simulink model "AFS_FinTabSim"  (R2026a)
settings: Solver=ode45  StopTime=P.sim.tStop  MaxStep=P.sim.maxStep  RelTol=1e-5
PostLoadFcn:
  | addpath(fileparts(get_param('AFS_FinTabSim','FileName')));
  | if ~evalin('base','exist(''P'',''var'')'), assignin('base','P',afs_params()); end
InitFcn:
  | if ~exist('P','var'), P = afs_params(); end
values from neighbouring files (symbols this model uses):
  P = afs_params()    [build_AFS_FinTabSim.m]    (also in run_AFS_FinTabSim.m)
libraries: simulink x4
settings Model: Creator=lando  LastModifiedBy=lando

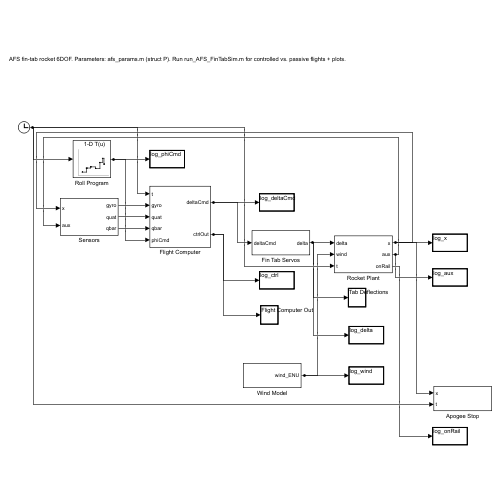
[thumbnail: Simulink's stored preview of the top-level diagram]
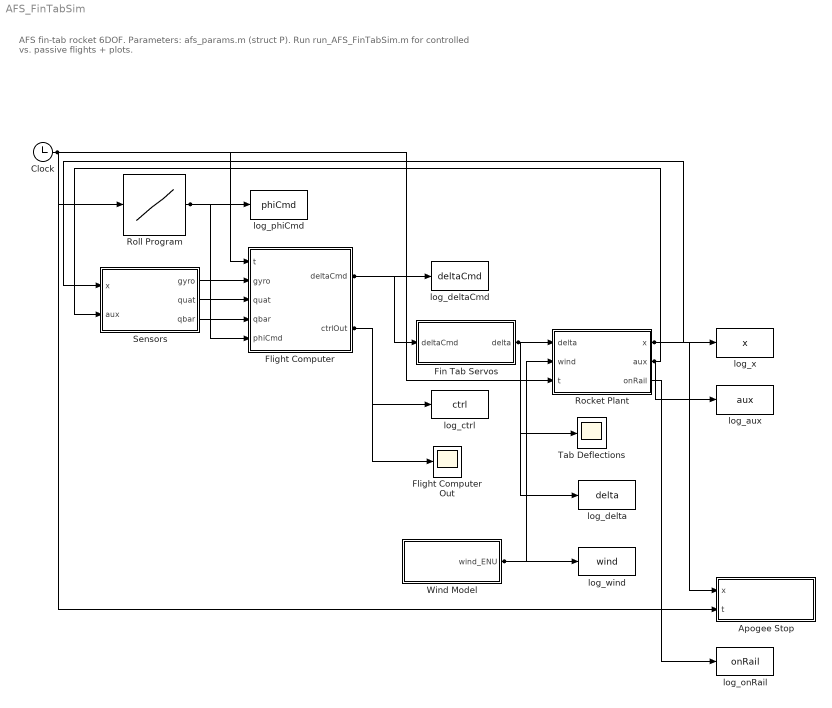
== system AFS_FinTabSim ==
  note: AFS fin-tab rocket 6DOF. Parameters: afs_params.m (struct P). Run run_AFS_FinTabSim.m for controlled vs. passive flights + plots.
  Apogee Stop : Subsystem
  Clock : Clock
  Fin Tab Servos : Subsystem
  Flight Computer : Subsystem
  Flight Computer Out : Scope
  Rocket Plant : Subsystem
  Roll Program : Lookup_n-D  NumberOfTableDimensions=1  BreakpointsForDimension1=P.ctrl.rollProg.t  Table=P.ctrl.rollProg.phi  InterpMethod=Flat  ExtrapMethod=Clip  InternalRulePriority=Speed  RndMeth=Simplest
  Sensors : Subsystem
  Tab Deflections : Scope
  Wind Model : Subsystem
  log_aux : ToWorkspace  VariableName=aux  SaveFormat=Timeseries  SampleTime=-1
  log_ctrl : ToWorkspace  VariableName=ctrl  SaveFormat=Timeseries  SampleTime=-1
  log_delta : ToWorkspace  VariableName=delta  SaveFormat=Timeseries  SampleTime=-1
  log_deltaCmd : ToWorkspace  VariableName=deltaCmd  SaveFormat=Timeseries  SampleTime=-1
  log_onRail : ToWorkspace  VariableName=onRail  SaveFormat=Timeseries  SampleTime=-1
  log_phiCmd : ToWorkspace  VariableName=phiCmd  SaveFormat=Timeseries  SampleTime=-1
  log_wind : ToWorkspace  VariableName=wind  SaveFormat=Timeseries  SampleTime=-1
  log_x : ToWorkspace  VariableName=x  SaveFormat=Timeseries  SampleTime=-1
  wires:
  Clock/1 -> Rocket Plant/3(t), Flight Computer/1(t), Apogee Stop/2(t), Roll Program/1
  Rocket Plant/3(onRail) -> log_onRail/1
  Roll Program/1 -> Flight Computer/5(phiCmd), log_phiCmd/1
  Sensors/3(qbar) -> Flight Computer/4(qbar)
  Sensors/2(quat) -> Flight Computer/3(quat)
  Sensors/1(gyro) -> Flight Computer/2(gyro)
  Flight Computer/2(ctrlOut) -> log_ctrl/1, Flight Computer Out/1
  Flight Computer/1(deltaCmd) -> Fin Tab Servos/1(deltaCmd), log_deltaCmd/1
  Fin Tab Servos/1(delta) -> Rocket Plant/1(delta), log_delta/1, Tab Deflections/1
  Wind Model/1(wind_ENU) -> Rocket Plant/2(wind), log_wind/1
  Rocket Plant/1(x) -> Apogee Stop/1(x), Sensors/1(x), log_x/1
  Rocket Plant/2(aux) -> Sensors/2(aux), log_aux/1

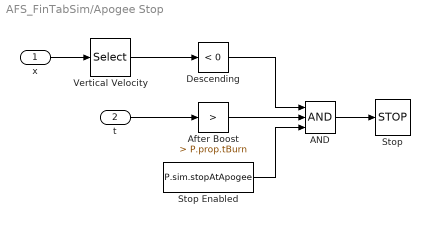
== system AFS_FinTabSim/Apogee Stop ==
  x : Inport
  t : Inport  Port=2
  AND : Logic  Inputs=3  AllPortsSameDT=off  OutDataTypeStr=boolean
  After Boost : simulink/Logic and Bit Operations/Compare To Constant  relop=>  const=P.prop.tBurn  OutDataTypeStr=boolean
  Descending : simulink/Logic and Bit Operations/Compare To Constant  relop=<  const=0  OutDataTypeStr=boolean
  Stop : Stop
  Stop Enabled : Constant  Value=P.sim.stopAtApogee  OutDataTypeStr=boolean
  Vertical Velocity : Selector  InputPortWidth=13  IndexOptions=Index vector (dialog)  Indices=6  OutputSizes=1
  wires:
  t/1 -> After Boost/1
  Vertical Velocity/1 -> Descending/1
  x/1 -> Vertical Velocity/1
  After Boost/1 -> AND/2
  Descending/1 -> AND/1
  AND/1 -> Stop/1
  Stop Enabled/1 -> AND/3

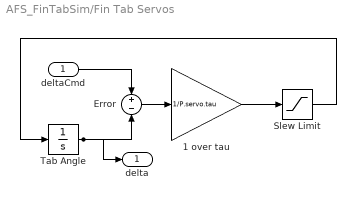
== system AFS_FinTabSim/Fin Tab Servos ==
  deltaCmd : Inport
  1 over tau : Gain  Gain=1/P.servo.tau
  Error : Sum  Inputs=+-
  Slew Limit : Saturate  UpperLimit=P.servo.rateMax  LowerLimit=-P.servo.rateMax
  Tab Angle : Integrator  InitialCondition=zeros(P.geo.nFins,1)  LimitOutput=on  UpperSaturationLimit=P.servo.defMax  LowerSaturationLimit=-P.servo.defMax
  delta : Outport
  wires:
  deltaCmd/1 -> Error/1
  Slew Limit/1 -> Tab Angle/1
  1 over tau/1 -> Slew Limit/1
  Tab Angle/1 -> Error/2, delta/1
  Error/1 -> 1 over tau/1

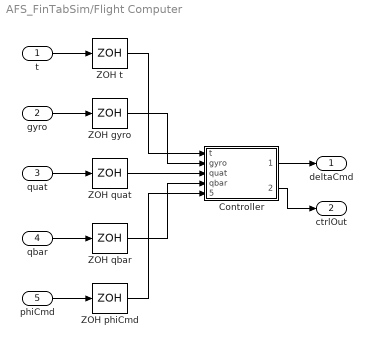
== system AFS_FinTabSim/Flight Computer ==
  t : Inport
  gyro : Inport  Port=2
  quat : Inport  Port=3
  qbar : Inport  Port=4
  phiCmd : Inport  Port=5
  Controller : MATLAB Function  TreatAsAtomicUnit=on
  ZOH gyro : ZeroOrderHold  SampleTime=P.sens.Ts
  ZOH phiCmd : ZeroOrderHold  SampleTime=P.sens.Ts
  ZOH qbar : ZeroOrderHold  SampleTime=P.sens.Ts
  ZOH quat : ZeroOrderHold  SampleTime=P.sens.Ts
  ZOH t : ZeroOrderHold  SampleTime=P.sens.Ts
  deltaCmd : Outport
  ctrlOut : Outport  Port=2
  wires:
  t/1 -> ZOH t/1
  ZOH gyro/1 -> Controller/2(gyro)
  ZOH t/1 -> Controller/1(t)
  quat/1 -> ZOH quat/1
  gyro/1 -> ZOH gyro/1
  ZOH quat/1 -> Controller/3(quat)
  phiCmd/1 -> ZOH phiCmd/1
  qbar/1 -> ZOH qbar/1
  ZOH qbar/1 -> Controller/4(qbar)
  ZOH phiCmd/1 -> Controller/5(phiCmd)
  Controller/1(deltaCmd) -> deltaCmd/1
  Controller/2(ctrlOut) -> ctrlOut/1

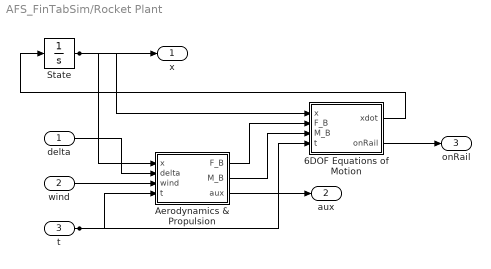
== system AFS_FinTabSim/Rocket Plant ==
  delta : Inport
  wind : Inport  Port=2
  t : Inport  Port=3
  6DOF Equations of Motion : MATLAB Function  TreatAsAtomicUnit=on
  Aerodynamics & Propulsion : MATLAB Function  TreatAsAtomicUnit=on
  State : Integrator  InitialCondition=P.x0
  x : Outport
  aux : Outport  Port=2
  onRail : Outport  Port=3
  wires:
  State/1 -> 6DOF Equations of Motion/1(x), Aerodynamics & Propulsion/1(x), x/1
  wind/1 -> Aerodynamics & Propulsion/3(wind)
  Aerodynamics & Propulsion/1(F_B) -> 6DOF Equations of Motion/2(F_B)
  t/1 -> Aerodynamics & Propulsion/4(t), 6DOF Equations of Motion/4(t)
  delta/1 -> Aerodynamics & Propulsion/2(delta)
  Aerodynamics & Propulsion/3(aux) -> aux/1
  Aerodynamics & Propulsion/2(M_B) -> 6DOF Equations of Motion/3(M_B)
  6DOF Equations of Motion/1(xdot) -> State/1
  6DOF Equations of Motion/2(onRail) -> onRail/1

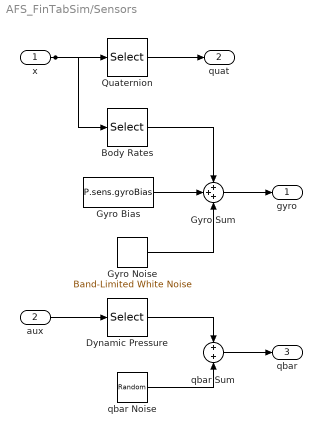
== system AFS_FinTabSim/Sensors ==
  x : Inport
  aux : Inport  Port=2
  Body Rates : Selector  InputPortWidth=13  IndexOptions=Index vector (dialog)  Indices=[11 12 13]  OutputSizes=1
  Dynamic Pressure : Selector  InputPortWidth=8  IndexOptions=Index vector (dialog)  Indices=4  OutputSizes=1
  Gyro Bias : Constant  Value=P.sens.gyroBias
  Gyro Noise : simulink/Sources/Band-Limited White Noise  Cov=P.sens.gyroNoise*[1 1 1]  Ts=P.sens.Ts  seed=P.sens.gyroSeed
  Gyro Sum : Sum  Inputs=+++
  Quaternion : Selector  InputPortWidth=13  IndexOptions=Index vector (dialog)  Indices=[7 8 9 10]  OutputSizes=1
  qbar Noise : RandomNumber  Variance=P.sens.qbarNoise^2  Seed=31  SampleTime=P.sens.Ts
  qbar Sum : Sum
  gyro : Outport
  quat : Outport  Port=2
  qbar : Outport  Port=3
  wires:
  Dynamic Pressure/1 -> qbar Sum/1
  Body Rates/1 -> Gyro Sum/1
  Gyro Bias/1 -> Gyro Sum/2
  Quaternion/1 -> quat/1
  aux/1 -> Dynamic Pressure/1
  x/1 -> Body Rates/1, Quaternion/1
  Gyro Sum/1 -> gyro/1
  qbar Noise/1 -> qbar Sum/2
  Gyro Noise/1 -> Gyro Sum/3
  qbar Sum/1 -> qbar/1

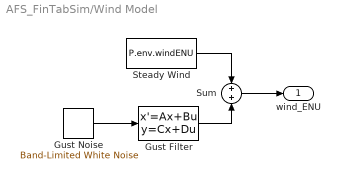
== system AFS_FinTabSim/Wind Model ==
  Gust Filter : StateSpace  A=-eye(3)/P.env.gustTau  B=eye(3)/P.env.gustTau  C=eye(3)  D=zeros(3)  InitialCondition=0
  Gust Noise : simulink/Sources/Band-Limited White Noise  Cov=P.env.gustPower*[1 1 0.3]  Ts=0.05  seed=P.env.gustSeed
  Steady Wind : Constant  Value=P.env.windENU
  Sum : Sum
  wind_ENU : Outport
  wires:
  Gust Noise/1 -> Gust Filter/1
  Steady Wind/1 -> Sum/1
  Gust Filter/1 -> Sum/2
  Sum/1 -> wind_ENU/1

== matlab function AFS_FinTabSim/Rocket Plant/Aerodynamics & Propulsion ==
  data: x input; F_B output; delta input; wind input; t input; M_B output; aux output; P parameter
function [F_B, M_B, aux] = fcn(x, delta, wind, t, P)
% Body-frame forces/moments: thrust, drag, body lift, fins, fin tabs.
% aux = [alpha; beta; mach; qbar; aoaTotal; thrust; mass; xCg]
[F_B, M_B, aux] = afs_aero(P, x, delta, wind, t);

== matlab function AFS_FinTabSim/Flight Computer/Controller ==
  data: t input; deltaCmd output; gyro input; quat input; qbar input; phiCmd input; ctrlOut output; P parameter
function [deltaCmd, ctrlOut] = fcn(t, gyro, quat, qbar, phiCmd, P)
% Fin-tab flight control law (see afs_controller.m). Runs at P.sens.Ts.
[deltaCmd, ctrlOut] = afs_controller(P, t, gyro, quat, qbar, phiCmd);

== matlab function AFS_FinTabSim/Rocket Plant/6DOF Equations of Motion ==
  data: x input; xdot output; F_B input; M_B input; t input; onRail output; P parameter
function [xdot, onRail] = fcn(x, F_B, M_B, t, P)
% Translational + rotational dynamics, quaternion kinematics, rail constraint.
[xdot, onRail] = afs_eom(P, x, F_B, M_B, t);
